simulink model "EMT_ML.before_diagnostic_fixes"  (R2024b)
settings: Solver=ode5  StartTime=0.0  StopTime=200  FixedStep=0.002  RelTol=1e-3
model workspace (MAT data in the model file):
  A = 7.3
  B = 2.71
  C0_shift = 200
  C1_shift = 200
  C2_shift = 200
  Cb = 70
  Cd = 0.6
  EMSInputBus : Simulink.Bus (value not decoded)
  Fb_max = 247500
  JA = 0.4
  JB = 0.4
  JZ = 0.4
  Jc1r2 = 0.01
  Jc3r4 = 0.01
  Jc4 = 0.01
  Je = 2.5
  Jh = 0.01
  Jq1 = 0.01
  Jq2 = 0.01
  Jr1 = 0.01
  Jr3s4 = 0.01
  Js123 = 0.01
  L = 4.472
  NE = [1600 1600 1600 1600 1600 1600 1600 1600 1600 1600 1600 1600 ... (840 elements, 30x28)]
  N_Te = 30
  N_ne = 28
  PE = [0 100.366530527 133.710336161 167.221698607 195.706356687 221.845219395 250.497434286 278.144308305 305.288511886 330.086920096 352.87464656 374.489475338 ... (840 elements, 30x28)]
  PN0 = 0
  Pb_epr = [-45 -45 -40 -30 0 30 40 45 45]
  Pb_max = [0 40 45 45 45]
  Pb_min = [-45 -45 -45 -40 0]
  Pe_ass = 230
  Pe_max = 1103
  Peg = [0 100 120 140 160 180 200 220 240 260 280 300 ... (53 elements, 1x53)]
  R_map = [0.09 0.089 0.09 0.091 0.092 0.093 0.094 0.095 0.096 0.097 0.098]
  SF_C0 = 1.5
  SF_C1 = 1.5
  SF_C2 = 1.5
  SF_Z1 = 1.5
  SF_Z2 = 1.5
  SF_ZD = 1.5
  SOC0 = 60
  SOC_epr = [30 31 50 59 60 61 70 79 80]
  SOC_map = [0 10 20 30 40 50 60 70 80 90 100]
  TA_max_map = [588.855 593.803361345 598.83559322 603.953846154 609.160344828 614.457391304 619.847368421 625.332743363 630.916071429 636.6 642.387272727 648.280733945 ... (115 elements, 1x115)]
  TA_min_map = [-588.855 -593.803361345 -598.83559322 -603.953846154 -609.160344828 -614.457391304 -619.847368421 -625.332743363 -630.916071429 -636.6 -642.387272727 -648.280733945 ... (115 elements, 1x115)]
  TAf = 0
  TB_max_map = [588.855 593.803361345 598.83559322 603.953846154 609.160344828 614.457391304 619.847368421 625.332743363 630.916071429 636.6 642.387272727 648.280733945 ... (115 elements, 1x115)]
  TB_min_map = [-588.855 -593.803361345 -598.83559322 -603.953846154 -609.160344828 -614.457391304 -619.847368421 -625.332743363 -630.916071429 -636.6 -642.387272727 -648.280733945 ... (115 elements, 1x115)]
  TBf = 0
  TE = [0 599 798 998 1168 1324 1495 1660 1822 1970 2106 2235 ... (840 elements, 30x28)]
  TS_A = 0.2
  TS_B = 0.2
  TS_C0 = 0.2
  TS_C1 = 0.2
  TS_C2 = 0.2
  TS_Z = 0.2
  TS_Z1 = 0.2
  TS_Z2 = 0.2
  TS_ZD = 0.2
  TZ_max_map = [537.13125 540.509433962 543.930379747 547.394904459 550.903846154 554.458064516 558.058441558 561.705882353 565.401315789 569.145695364 572.94 576.785234899 ... (131 elements, 1x131)]
  TZ_min_map = [-537.13125 -540.509433962 -543.930379747 -547.394904459 -550.903846154 -554.458064516 -558.058441558 -561.705882353 -565.401315789 -569.145695364 -572.94 -576.785234899 ... (131 elements, 1x131)]
  TZf = 0
  T_generator = [0 185 493.333333333 801.666666667 1110 1418.33333333 1726.66666667]
  T_motor = [0 185 493.333333333 801.666666667 1110 1418.33333333 1726.66666667]
  Te_map = [0 599 798 998 1168 1324 1495 1660 1822 1970 2106 2235 ... (30 elements, 1x30)]
  Te_max = 2754
  Te_max_map = [1168 1324 1495 1660 1822 1970 2106 2235 2355 2458 2543 2606 ... (28 elements, 1x28)]
  Te_start = 1600
  Tef = 100
  Teg = [0 596.8125 636.6 718.741935484 799.916230366 859.41 954.422788606 954.9 996.417391304 1078.98305085 1114.05 1169.26530612 ... (53 elements, 1x53)]
  Temax = 998
  Time = [0 0.1 0.2 0.3 0.4 0.5 0.6 0.7 0.8 0.9 1 1.1 ... (2001 elements, 1x2001)]
  Time_ele = [0 4 8 12 16 20 24 28 32 36 40 44 ... (401 elements, 1x401)]
  Time_fg = [0 2 4 6 8 10 12 14 16 18 20 22 ... (801 elements, 1x801)]
  Tmax_C0 = 2754
  Tmax_C1 = 3505.25455609
  Tmax_C2 = 3505.25455609
  Tmax_Z1 = 5584.80955498
  Tmax_Z2 = 16307.6439005
  Tmax_ZD = 3855.6
  Ts_e = 0.1
  Uoc_map = [814.5 917 933.25 945.75 958.25 969.25 978 985.25 993.25 1003.25 1050]
  V_Shift12 = 32
  V_Shift21 = 25
  V_Start = 10
  Voltage0 = 900
  Voltage_epr = [750 760 900 1000 1050]
  Y_engine = 0.955
  Yc = 0.98
  Yh = 0.96
  Yo = 0.92
  Yq = 0.94
  Z1_shift = 200
  Z2_shift = 200
  a11 = 1.54241568346
  a11_L = 1.54241568346
  a12 = -3.86074191629
  a12_L = 2.43173643789
  a21 = -1.04963112005
  a22 = 2.46948356808
  b11 = 0
  b11_L = 0
  b12 = 3.33
  b12_L = 7.8036
  b21 = 2.23571428571
  b22 = -2.13
  c11 = -0.648333656565
  c12 = 0
  c21 = -0.648333656565
  c22 = 0.680511182109
  controller_id = 1
  controller_name = 'Existing heuristic-grid EMS'
  cycle_grade = [0 0 0 0 0 0 0 0 0 0 0 0 ... (2001 elements, 1x2001)]
  cycle_road = [0.045 0.045 0.045 0.045 0.045 0.045 0.045 0.045 0.045 0.045 0.045 0.045 ... (2001 elements, 1x2001)]
  cycle_steering = [0 0 0 0 0 0 0 0 0 0 0 0 ... (2001 elements, 1x2001)]
  cycle_time = [0 0.1 0.2 0.3 0.4 0.5 0.6 0.7 0.8 0.9 1 1.1 ... (2001 elements, 1x2001)]
  d11 = -0.751666343435
  d12 = 0.3003003003
  d21 = -0.751666343435
  d22 = 0.319488817891
  e11 = -1.54241568346
  e12 = 0
  e21 = 1.04963112005
  e22 = -2.23571428571
  eff_generator = [0.8 0.8 0.79 0.79 0.76 0.74 0.72 0.8 0.85 0.88 0.85 0.8 ... (84 elements, 7x12)]
  eff_motor = [0.8 0.8 0.79 0.79 0.76 0.74 0.72 0.8 0.85 0.88 0.85 0.8 ... (84 elements, 7x12)]
  ele_map = [10 11.46 14.13 19.24 20.94 23.21 20.29 20.23 22.28 17.66 16.24 18.95 ... (401 elements, 1x401)]
  ems_runtime_config : object (value not decoded)
  f11 = -3.86074191629
  f12 = 3.33
  f21 = 2.46948356808
  f22 = -2.13
  fg = 0.045
  fg_map = [0.0125 0.0215 0.0332 0.0452 0.0525 0.0589 0.0584 0.0592 0.0621 0.0576 0.055 0.0572 ... (801 elements, 1x801)]
  fuel_gpkwh = [269.874826377 269.874826377 260.084605263 254.895150301 249.802821062 244.062054381 234.972466555 226.630558735 223.93243551 227.612775381 231.379615385 228.983738255 ... (840 elements, 30x28)]
  fuel_map = [269.874826377 269.874826377 260.084605263 254.895150301 249.802821062 244.062054381 234.972466555 226.630558735 223.93243551 227.612775381 231.379615385 228.983738255 ... (840 elements, 30x28)]
  fuel_map_N = [269.874826377 269.874826377 260.084605263 254.895150301 249.802821062 nan nan nan nan nan nan nan ... (840 elements, 30x28)]
  i = 28
  ic = 4.42
  iq = 1.4
  it = 4
  j = 30
  k1 = 2.13
  k2 = 2.13
  k3 = 2.33
  k4 = 1.92
  kh = 2.88
  kq = 2.17
  kt = 1.83
  mass = 45000
  miu_max = 0.8
  nA_map = [-6000 -5950 -5900 -5850 -5800 -5750 -5700 -5650 -5600 -5550 -5500 -5450 ... (115 elements, 1x115)]
  nA_max = 6000
  nA_min = -6000
  nB_map = [-6000 -5950 -5900 -5850 -5800 -5750 -5700 -5650 -5600 -5550 -5500 -5450 ... (115 elements, 1x115)]
  nB_max = 6000
  nB_min = -6000
  nB_start = 0
  nZ_map = [-8000 -7950 -7900 -7850 -7800 -7750 -7700 -7650 -7600 -7550 -7500 -7450 ... (131 elements, 1x131)]
  nZ_max = 8000
  nZ_min = -8000
  n_generator = [0 318.5 796.25 1274 1751.75 2229.5 2707.25 3185 3662.75 4140.5 4618.25 7007]
  n_motor = [0 318.5 796.25 1274 1751.75 2229.5 2707.25 3185 3662.75 4140.5 4618.25 7007]
  ne_idl = 3000
  ne_map = [1600 1700 1800 1900 2000 2100 2200 2300 2400 2500 2600 2700 ... (28 elements, 1x28)]
  ne_max = 4200
  ne_min = 1600
  ne_start = 200
  neg = [1600 1600 1800 1860 1910 2000 2001 2200 2300 2301 2400 2450 ... (53 elements, 1x53)]
  no_Shift12 = 1589.43589002
  no_Shift21 = 1241.74678908
  rz = 0.318
  startup_feedback_delay_s = 0.002
  startup_power_share = 0.5
  startup_speed_regularizer_rpm = 100
  v_cyc = [0 0 0 0 0 0 0 0 0 0 0 0 ... (2001 elements, 1x2001)]
  voltage_HighA = 1050
  voltage_HighB = 1050
  voltage_HighZ = 1050
  voltage_LowA = 750
  voltage_LowB = 750
  voltage_LowZ = 750
symbols that are objects in the model workspace (value not decoded): ems_runtime_config
undefined symbols (not defined in the file or in its folder): sigbuilder_block
libraries: fl_lib x82, nesl_utility x55, simulink x49, sdl_lib x10, simulink_need_slupdate x6, powerlib_extras x1
(part 3 of 7)

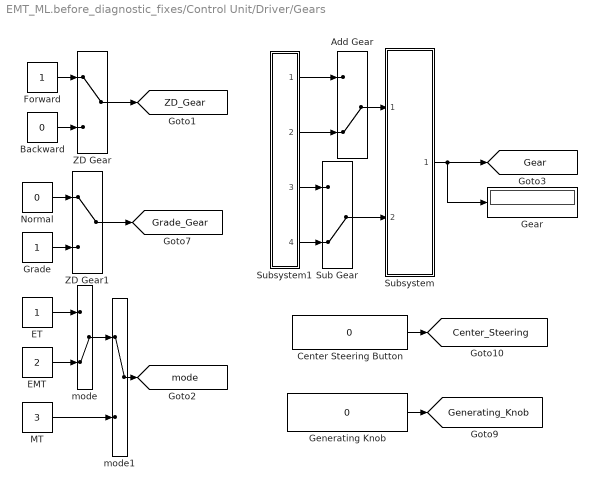
== system EMT_ML.before_diagnostic_fixes/Control Unit/Driver/Gears ==
  "Add Gear " : ManualSwitch  CurrentSetting=0
  Backward : Constant  Value=0
  Center Steering Button : Constant  Value=0
  EMT : Constant  Value=2
  ET : Constant
  Forward : Constant
  Gear : Display
  Generating Knob : Constant  Value=0
  Grade : Constant
  MT : Constant  Value=3
  Normal : Constant  Value=0
  Sub Gear : ManualSwitch  CurrentSetting=0
  Subsystem : Subsystem
  Subsystem1 : Subsystem
  ZD Gear : ManualSwitch
  ZD Gear1 : ManualSwitch
  mode : ManualSwitch  CurrentSetting=0
  mode1 : ManualSwitch
  tag scope: Center_Steering=global, Gear=global, Generating_Knob=global, Grade_Gear=global, ZD_Gear=global, mode=global
  wires:
  ZD Gear1/1 -> [Grade_Gear]
  Normal/1 -> ZD Gear1/1
  Grade/1 -> ZD Gear1/2
  Center Steering Button/1 -> [Center_Steering]
  Generating Knob/1 -> [Generating_Knob]
  mode/1 -> mode1/1
  mode1/1 -> [mode]
  MT/1 -> mode1/2
  EMT/1 -> mode/2
  Subsystem/1(Gear) -> [Gear], Gear/1
  Sub Gear/1 -> Subsystem/2(Sub)
  "Add Gear "/1 -> Subsystem/1(Add)
  Subsystem1/4(4) -> Sub Gear/2
  Subsystem1/3(3) -> Sub Gear/1
  Subsystem1/2(2) -> "Add Gear "/2
  Subsystem1/1(1) -> "Add Gear "/1
  ET/1 -> mode/1
  ZD Gear/1 -> [ZD_Gear]
  Forward/1 -> ZD Gear/1
  Backward/1 -> ZD Gear/2

== system EMT_ML.before_diagnostic_fixes/Control Unit/Driver/Grade Angle ==
  " 0.1" : ManualSwitch  CurrentSetting=0
  10 : ManualSwitch
  Add angle : ManualSwitch
  Forward : Constant  Value=32
  Forward1 : Lookup_n-D  NumberOfTableDimensions=1  BreakpointsForDimension1=cycle_time  Table=cycle_grade  InternalRulePriority=Speed  RndMeth=Simplest
  Forward1_clock : Clock
  Sub angle : ManualSwitch  CurrentSetting=0
  Subsystem4 : Subsystem  mask{Parameter1=on}
      mask prompts: Parameter1 "Pedal"
  Subsystem6 : Subsystem
  Transfer Fcn1 : TransferFcn  Denominator=[0.02 1]
  angle : Display
  tag scope: angle=global
  wires:
  Subsystem4/1(Out1) -> Add angle/1
  Subsystem4/2(Out2) -> Add angle/2
  Subsystem4/3(Out3) -> Sub angle/1
  Add angle/1 -> Subsystem6/1(Add)
  Sub angle/1 -> Subsystem6/2(Sub)
  Subsystem4/4(Out4) -> Sub angle/2
  Subsystem4/5(Out5) -> " 0.1"/1
  Subsystem4/6(Out6) -> " 0.1"/2
  Subsystem4/7(Out7) -> 10/1
  Subsystem4/8(Out8) -> 10/2
  " 0.1"/1 -> Subsystem6/3(0.1)
  10/1 -> Subsystem6/4(10)
  Subsystem6/1(angle) -> Transfer Fcn1/1, angle/1
  Forward1_clock/1 -> Forward1/1
  Forward1/1 -> [angle]

== system EMT_ML.before_diagnostic_fixes/Control Unit/Driver/Ground Resistance Coefficient ==
  *0.1 : ManualSwitch
  *10 : ManualSwitch
  Add : Sum
  Add fg : ManualSwitch  CurrentSetting=0
  Add1 : Sum
  Forward : Constant  Value=0.07
  Forward1 : Lookup_n-D  NumberOfTableDimensions=1  BreakpointsForDimension1=cycle_time  Table=cycle_road  InternalRulePriority=Speed  RndMeth=Simplest
  Forward1_clock : Clock
  Road : Subsystem
  Road1 : Subsystem
  Saturation : Saturate  UpperLimit=0.6  LowerLimit=0.04
  Saturation1 : Saturate  UpperLimit=0.6  LowerLimit=0.04
  Sub fg : ManualSwitch  CurrentSetting=0
  Subsystem2 : Subsystem  mask{Parameter1=on}
      mask prompts: Parameter1 "Pedal"
  Subsystem3 : Subsystem
  Transfer Fcn1 : TransferFcn  Denominator=[0.02 1]
  Uniform Random Number : UniformRandomNumber  Minimum=-0.01  Maximum=0.01  SampleTime=1
  fg : Display
  tag scope: fg_act=global
  wires:
  Road/1(fg) -> Add/2
  Subsystem3/1(fg) -> Add/1
  Subsystem2/1(Out1) -> Add fg/1
  Subsystem2/2(Out2) -> Add fg/2
  Subsystem2/3(Out3) -> Sub fg/1
  Add fg/1 -> Subsystem3/1(Add)
  Sub fg/1 -> Subsystem3/2(Sub)
  Subsystem2/4(Out4) -> Sub fg/2
  Subsystem2/5(Out5) -> *0.1/1
  Subsystem2/6(Out6) -> *0.1/2
  Subsystem2/7(Out7) -> *10/1
  Subsystem2/8(Out8) -> *10/2
  *0.1/1 -> Subsystem3/3(0.1)
  *10/1 -> Subsystem3/4(10)
  Transfer Fcn1/1 -> fg/1
  Add/1 -> Saturation/1
  Uniform Random Number/1 -> Add1/2
  Road1/1(fg) -> Saturation1/1
  Forward/1 -> Add1/1
  Add1/1 -> Transfer Fcn1/1
  Forward1_clock/1 -> Forward1/1
  Forward1/1 -> [fg_act]

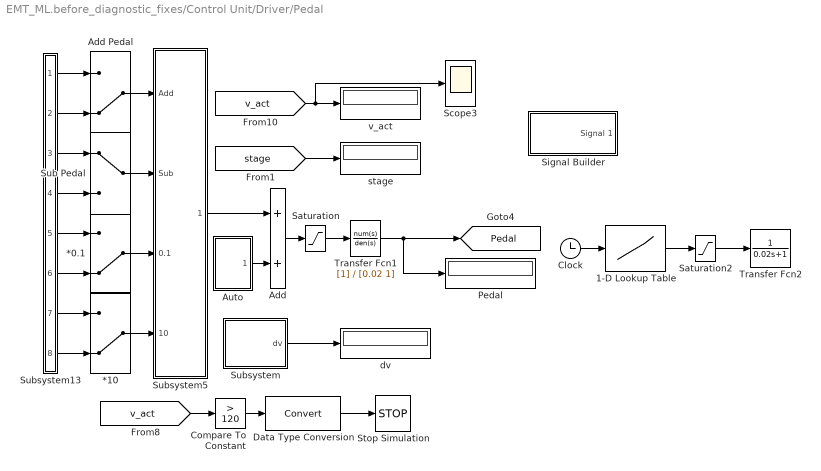
== system EMT_ML.before_diagnostic_fixes/Control Unit/Driver/Pedal  ==
  *0.1 : ManualSwitch  CurrentSetting=0
  *10 : ManualSwitch  CurrentSetting=0
  1-D Lookup Table : Lookup_n-D  NumberOfTableDimensions=1  BreakpointsForDimension1=[0 100 101 200]  Table=[1 1 -1 -1]  RndMeth=Simplest
  Add : Sum
  Add Pedal : ManualSwitch  CurrentSetting=0
  Auto : Subsystem
  Clock : Clock
  Compare To Constant : simulink/Logic and Bit Operations/Compare To Constant  relop=>  const=120  OutDataTypeStr=uint8
  Data Type Conversion : DataTypeConversion  SaturateOnIntegerOverflow=off  RndMeth=Floor
  Pedal : Display
  Saturation : Saturate  UpperLimit=1  LowerLimit=-1
  Saturation2 : Saturate  UpperLimit=1  LowerLimit=-1
  Scope3 : Scope
  Signal Builder : Subsystem  Tag=STV Subsys  LoadFcn=sigbuilder_block('load');  StartFcn=sigbuilder_block('start');  StopFcn=sigbuilder_block('stop');  ClipboardFcn=sigbuilder_block('clipboard');  mask(Sigbuilder block){tuvar=[0:10]}
      mask help: Simulink:masks:SigbuilderBlock_MD
      mask init:
      | if ~strcmp(get_param(bdroot(gcbh),'SimulationStatus'),'stopped') tuvar = sigbuilder_block('maskInit'); end
      settings: CopyFcn=sigbuilder_block('copy');  DeleteFcn=sigbuilder_block('delete');  ModelCloseFcn=sigbuilder_block('modelClose');  PreSaveFcn=sigbuilder_block('preSave');  PauseFcn=sigbuilder_block('pause')  ContinueFcn=sigbuilder_block('continue')  NameChangeFcn=sigbuilder_block('namechange');  OpenFcn=sigbuilder_block('open',[437.25 199.5 550.5 399.75 ]);  CloseFcn=sigbuilder_block('close');
      mask Display: plot(0, 0, 100, 100,[2, 2, 32, 32, 2], [68, 8, 8, 68, 68],[32, 2], [38, 38], [32, 19, 2],[53, 60, 44], [32, 17, 17, 2],[16, 16, 31, 31]);txt = getActiveGroup(gcbh);text(2, 100, txt,'verticalAlignment', 'top');
  Stop Simulation : Stop
  Sub Pedal : ManualSwitch
  Subsystem : Subsystem
  Subsystem13 : Subsystem  mask{Parameter1=on}
      mask prompts: Parameter1 "Pedal"
  Subsystem5 : Subsystem
  Transfer Fcn1 : TransferFcn  Denominator=[0.02 1]
  Transfer Fcn2 : TransferFcn  Denominator=[0.02 1]
  dv : Display
  stage : Display
  v_act : Display
  tag scope: Pedal=global
  wires:
  Subsystem5/1(Pedal) -> Add/1
  Subsystem/1(dv) -> dv/1
  [stage] -> stage/1
  [v_act] -> Scope3/1, v_act/1
  *10/1 -> Subsystem5/4(10)
  *0.1/1 -> Subsystem5/3(0.1)
  Subsystem13/8(Out8) -> *10/2
  Subsystem13/7(Out7) -> *10/1
  Subsystem13/6(Out6) -> *0.1/2
  Subsystem13/5(Out5) -> *0.1/1
  Subsystem13/4(Out4) -> Sub Pedal/2
  Sub Pedal/1 -> Subsystem5/2(Sub)
  Add Pedal/1 -> Subsystem5/1(Add)
  Subsystem13/3(Out3) -> Sub Pedal/1
  Subsystem13/2(Out2) -> Add Pedal/2
  Subsystem13/1(Out1) -> Add Pedal/1
  [v_act] -> Compare To Constant/1
  Compare To Constant/1 -> Data Type Conversion/1
  Data Type Conversion/1 -> Stop Simulation/1
  Saturation/1 -> Transfer Fcn1/1
  Add/1 -> Saturation/1
  Clock/1 -> 1-D Lookup Table/1
  1-D Lookup Table/1 -> Saturation2/1
  Saturation2/1 -> Transfer Fcn2/1
  Auto/1(Pedal) -> Add/2
  Transfer Fcn1/1 -> Pedal/1, [Pedal]

== system EMT_ML.before_diagnostic_fixes/Control Unit/Driver/Wheel Angle ==
  " x 0.1" : ManualSwitch  CurrentSetting=0
  Add wheel : ManualSwitch
  Sub Wheel : ManualSwitch  CurrentSetting=0
  Subsystem1 : Subsystem  mask{Parameter1=on}
      mask prompts: Parameter1 "Pedal"
  Subsystem2 : Subsystem
  Wheel : Display
  x10 : ManualSwitch
  tag scope: Wheel=global
  wires:
  Subsystem2/1(wheel) -> Wheel/1, [Wheel]
  Subsystem1/1(Out1) -> Add wheel/1
  Subsystem1/2(Out2) -> Add wheel/2
  Subsystem1/3(Out3) -> Sub Wheel/1
  Add wheel/1 -> Subsystem2/1(Add)
  Sub Wheel/1 -> Subsystem2/2(Sub)
  Subsystem1/4(Out4) -> Sub Wheel/2
  Subsystem1/5(Out5) -> " x 0.1"/1
  Subsystem1/6(Out6) -> " x 0.1"/2
  Subsystem1/7(Out7) -> x10/1
  Subsystem1/8(Out8) -> x10/2
  " x 0.1"/1 -> Subsystem2/3(0.1)
  x10/1 -> Subsystem2/4(10)

== system EMT_ML.before_diagnostic_fixes/Front Gear/C0/C0 ==
  Press : Inport
  C0 : sdl_lib/Clutches/Disc Friction Clutch  geometry_model=2  r_eff=130 mm  d_o=145*2 mm  d_i=110*2 mm  nS=6  piston_area=0.0347 m^2  unidirectional=0  friction_model=1  mu_w_vector=[ 0 0.1 0.2 0.3 0.4 0.5 1 2 5 10 100 1000 ] rad/s  temperature_TLU=[280.0, 300.0, 320.0] K  mu_static=0.10  mu_static_vector=[0.4, 0.38, 0.36]  mu_coulomb=0.06  mu_coulomb_vector=[ 0.29 0.28 0.26 0.22 0.21 0.2 0.2 0.19 0.19 0.19 0.19 0.19 ]  mu_coulomb_temp_vector=[0.3, 0.28, 0.25]  mu_coulomb_matrix=[0.34, 0.32, 0.3; 0.3, 0.28, 0.25; 0.25, 0.2, 0.15]  mu_interp_method=1  mu_extrap_method=1  d_f=0.6  w_tol=0.001 rad/s  pressure_min=1560 Pa  mu_visc=0.0256 N*m/(rad/s)  initial_state_locked=1  thermal_mass=25 kJ/K  T_init=300 K
      settings: InternalSimscapePortConfiguration="{\"Bottom\":[],\"Left\":[{\"id\":\"P\",\"label\":\"P\",\"type\":\"input\"},{\"id\":\"B\",\"label\":\"B\",\"type\":\"foundation.mechanical.rotational.rotational\"}],\"Right\":[{\"id\":\"F\",\"label\":\"F\",\"type\":\"foundation.mechanical.rotational.rotational\"}],\"Top\":[]}"
  Simulink-PS Converter : nesl_utility/Simulink-PS Converter  PhysicalDomain=network_engine_domain  SubClassName=ps_input  LeftPortType=input  RightPortType=output  PseudoPeriodic=off  Frequencies=[]  NoiseDistribution=none  NoiseParameters=[]  Unit=Pa  AffineConversion=off  FilteringAndDerivatives=filter  SimscapeFilterOrder=1  InputFilterTimeConstant=.001  UdotUserProvided=1
  Slip Sensor : Subsystem  mask(Slip Sensor){}
      mask help: The speed unit is r/min.
  Tire Radius2 : Gain  Gain=2500000
  In : PMIOPort  Side=Left
  Out : PMIOPort  Port=2  Side=Right
  r/min : Outport
  wires:
  Slip Sensor/1(r/min) -> r/min/1
  Press/1 -> Tire Radius2/1
  Tire Radius2/1 -> Simulink-PS Converter/1
  connections:
  Slip Sensor/LConn1 -- C0/LConn2 -- In/RConn1
  Slip Sensor/RConn1 -- C0/RConn1 -- Out/RConn1
  Simulink-PS Converter/RConn1 -- C0/LConn1

== system EMT_ML.before_diagnostic_fixes/Front Gear/C0/Power ==
  Gain1 : Gain  Gain=1/9549
  Product3 : Product  RndMeth=Zero
  Speed Sensor : Subsystem  mask(Speed Sensor){}
      mask help: The speed unit is r/min.
  Torque Sensor : Subsystem  mask(Torque Sensor){}
      mask help: The torque unit is Nm.
  In : PMIOPort  Side=Left
  Out : PMIOPort  Port=2  Side=Right
  kW : Outport
  wires:
  Speed Sensor/1(r/min) -> Product3/2
  Torque Sensor/1(Nm) -> Gain1/1
  Gain1/1 -> Product3/1
  Product3/1 -> kW/1
  connections:
  Out/RConn1 -- Torque Sensor/RConn1 -- Speed Sensor/LConn1
  In/RConn1 -- Torque Sensor/LConn1

== system EMT_ML.before_diagnostic_fixes/Front Gear/C0/Power1 ==
  Gain1 : Gain  Gain=1/9549
  Product3 : Product  RndMeth=Zero
  Speed Sensor : Subsystem  mask(Speed Sensor){}
      mask help: The speed unit is r/min.
  Torque Sensor : Subsystem  mask(Torque Sensor){}
      mask help: The torque unit is Nm.
  In : PMIOPort  Side=Left
  Out : PMIOPort  Port=2  Side=Right
  kW : Outport
  wires:
  Product3/1 -> kW/1
  Gain1/1 -> Product3/1
  Torque Sensor/1(Nm) -> Gain1/1
  Speed Sensor/1(r/min) -> Product3/2
  connections:
  In/RConn1 -- Torque Sensor/LConn1
  Torque Sensor/RConn1 -- Out/RConn1 -- Speed Sensor/LConn1

== system EMT_ML.before_diagnostic_fixes/Front Gear/Subsystem/Speed Sensor ==
  Ideal Rotational Motion Sensor : fl_lib/Mechanical/Mechanical Sensors/Ideal Rotational Motion Sensor  reference=foundation.enum.MeasurementReference.difference  acceleration_port=false  velocity_port=true  position_port=true  wrap_angle=false  offset=0 rad
  PS-Simulink Converter : nesl_utility/PS-Simulink Converter  PhysicalDomain=network_engine_domain  SubClassName=ps_output  LeftPortType=input  RightPortType=output  PseudoPeriodic=off  Frequencies=[]  VectorFormat=1-D array  Unit=rad/s  AffineConversion=off
  Reference : fl_lib/Mechanical/Rotational Elements/Mechanical Rotational Reference
  Tire Radius2 : Gain  Gain=30/pi
  shaft : PMIOPort  Side=Left
  r/min : Outport
  wires:
  Tire Radius2/1 -> r/min/1
  PS-Simulink Converter/1 -> Tire Radius2/1
  connections:
  shaft/RConn1 -- Ideal Rotational Motion Sensor/LConn1
  Reference/LConn1 -- Ideal Rotational Motion Sensor/RConn1
  PS-Simulink Converter/LConn1 -- Ideal Rotational Motion Sensor/RConn2

== system EMT_ML.before_diagnostic_fixes/Front Gear/Subsystem/Torque Sensor ==
  Ideal Torque Sensor : fl_lib/Mechanical/Mechanical Sensors/Ideal Torque Sensor
  PS-Simulink Converter : nesl_utility/PS-Simulink Converter  PhysicalDomain=network_engine_domain  SubClassName=ps_output  LeftPortType=input  RightPortType=output  PseudoPeriodic=off  Frequencies=[]  VectorFormat=1-D array  Unit=1  AffineConversion=off
  In : PMIOPort  Side=Left
  Out : PMIOPort  Port=2  Side=Right
  Nm : Outport
  wires:
  PS-Simulink Converter/1 -> Nm/1
  connections:
  PS-Simulink Converter/LConn1 -- Ideal Torque Sensor/RConn2
  In/RConn1 -- Ideal Torque Sensor/LConn1
  Ideal Torque Sensor/RConn1 -- Out/RConn1

== system EMT_ML.before_diagnostic_fixes/Power Coupler /C1/C2 ==
  Press : Inport
  C1 : sdl_lib/Clutches/Disc Friction Clutch  geometry_model=2  r_eff=130 mm  d_o=167*2 mm  d_i=143*2 mm  nS=8  piston_area=0.0290 m^2  unidirectional=0  friction_model=1  mu_w_vector=[ 0 0.1 0.2 0.3 0.4 0.5 1 2 5 10 100 1000 ] rad/s  temperature_TLU=[280.0, 300.0, 320.0] K  mu_static=0.10  mu_static_vector=[0.4, 0.38, 0.36]  mu_coulomb=0.06  mu_coulomb_vector=[ 0.29 0.28 0.26 0.22 0.21 0.2 0.2 0.19 0.19 0.19 0.19 0.19 ]  mu_coulomb_temp_vector=[0.3, 0.28, 0.25]  mu_coulomb_matrix=[0.34, 0.32, 0.3; 0.3, 0.28, 0.25; 0.25, 0.2, 0.15]  mu_interp_method=1  mu_extrap_method=1  d_f=0.6  w_tol=0.001 rad/s  pressure_min=1840 Pa  mu_visc=0.0414 N*m/(rad/s)  initial_state_locked=0  thermal_mass=25 kJ/K  T_init=300 K
      settings: InternalSimscapePortConfiguration="{\"Bottom\":[],\"Left\":[{\"id\":\"P\",\"label\":\"P\",\"type\":\"input\"},{\"id\":\"B\",\"label\":\"B\",\"type\":\"foundation.mechanical.rotational.rotational\"}],\"Right\":[{\"id\":\"F\",\"label\":\"F\",\"type\":\"foundation.mechanical.rotational.rotational\"}],\"Top\":[]}"
  Simulink-PS Converter : nesl_utility/Simulink-PS Converter  PhysicalDomain=network_engine_domain  SubClassName=ps_input  LeftPortType=input  RightPortType=output  PseudoPeriodic=off  Frequencies=[]  NoiseDistribution=none  NoiseParameters=[]  Unit=Pa  AffineConversion=off  FilteringAndDerivatives=filter  SimscapeFilterOrder=1  InputFilterTimeConstant=.001  UdotUserProvided=1
  Slip Sensor : Subsystem  mask(Slip Sensor){}
      mask help: The speed unit is r/min.
  Tire Radius2 : Gain  Gain=2500000
  In : PMIOPort  Side=Left
  Out : PMIOPort  Port=2  Side=Right
  r/min : Outport
  wires:
  Tire Radius2/1 -> Simulink-PS Converter/1
  Press/1 -> Tire Radius2/1
  Slip Sensor/1(r/min) -> r/min/1
  connections:
  Simulink-PS Converter/RConn1 -- C1/LConn1
  In/RConn1 -- C1/LConn2 -- Slip Sensor/LConn1
  C1/RConn1 -- Out/RConn1 -- Slip Sensor/RConn1

== system EMT_ML.before_diagnostic_fixes/Power Coupler /C1/Power ==
  Gain1 : Gain  Gain=1/9549
  Product3 : Product  RndMeth=Zero
  Speed Sensor : Subsystem  mask(Speed Sensor){}
      mask help: The speed unit is r/min.
  Torque Sensor : Subsystem  mask(Torque Sensor){}
      mask help: The torque unit is Nm.
  In : PMIOPort  Side=Left
  Out : PMIOPort  Port=2  Side=Right
  kW : Outport
  wires:
  Product3/1 -> kW/1
  Gain1/1 -> Product3/1
  Torque Sensor/1(Nm) -> Gain1/1
  Speed Sensor/1(r/min) -> Product3/2
  connections:
  In/RConn1 -- Torque Sensor/LConn1
  Torque Sensor/RConn1 -- Out/RConn1 -- Speed Sensor/LConn1

== system EMT_ML.before_diagnostic_fixes/Power Coupler /C1/Power1 ==
  Gain1 : Gain  Gain=1/9549
  Product3 : Product  RndMeth=Zero
  Speed Sensor : Subsystem  mask(Speed Sensor){}
      mask help: The speed unit is r/min.
  Torque Sensor : Subsystem  mask(Torque Sensor){}
      mask help: The torque unit is Nm.
  In : PMIOPort  Side=Left
  Out : PMIOPort  Port=2  Side=Right
  kW : Outport
  wires:
  Speed Sensor/1(r/min) -> Product3/2
  Torque Sensor/1(Nm) -> Gain1/1
  Gain1/1 -> Product3/1
  Product3/1 -> kW/1
  connections:
  Speed Sensor/LConn1 -- Out/RConn1 -- Torque Sensor/RConn1
  In/RConn1 -- Torque Sensor/LConn1

== system EMT_ML.before_diagnostic_fixes/Power Coupler /Z1/Z ==
  Abs : Abs  SaturateOnIntegerOverflow=off
  Add : Sum  Inputs=+-
  Power : Subsystem
  Power1 : Subsystem
  Z1 : Subsystem
  In : PMIOPort  Side=Left
  Out : PMIOPort  Port=2  Side=Right
  tag scope: Z1_loss=global, Z1_rela=global
  wires:
  Z1/1(r/min) -> [Z1_rela]
  [Press_Z1] -> Z1/1(Press)
  Power1/1(kW) -> Add/2
  Power/1(kW) -> Add/1
  Abs/1 -> [Z1_loss]
  Add/1 -> Abs/1
  connections:
  In/RConn1 -- Power/LConn1
  Power/RConn1 -- Z1/LConn1
  Z1/RConn1 -- Power1/LConn1
  Power1/RConn1 -- Out/RConn1

== system EMT_ML.before_diagnostic_fixes/Power Coupler /Z2/Z ==
  Abs : Abs  SaturateOnIntegerOverflow=off
  Add : Sum  Inputs=+-
  Power : Subsystem
  Power1 : Subsystem
  Z2 : Subsystem
  In : PMIOPort  Side=Left
  Out : PMIOPort  Port=2  Side=Right
  tag scope: Z2_loss=global, Z2_rela=global
  wires:
  [Press_Z2] -> Z2/1(Press)
  Z2/1(r/min) -> [Z2_rela]
  Add/1 -> Abs/1
  Abs/1 -> [Z2_loss]
  Power1/1(kW) -> Add/2
  Power/1(kW) -> Add/1
  connections:
  In/RConn1 -- Power/LConn1
  Power/RConn1 -- Z2/LConn1
  Z2/RConn1 -- Power1/LConn1
  Power1/RConn1 -- Out/RConn1

== system EMT_ML.before_diagnostic_fixes/Rear Gear/Subsystem/Speed Sensor ==
  Ideal Rotational Motion Sensor : fl_lib/Mechanical/Mechanical Sensors/Ideal Rotational Motion Sensor  reference=foundation.enum.MeasurementReference.difference  acceleration_port=false  velocity_port=true  position_port=true  wrap_angle=false  offset=0 rad
  PS-Simulink Converter : nesl_utility/PS-Simulink Converter  PhysicalDomain=network_engine_domain  SubClassName=ps_output  LeftPortType=input  RightPortType=output  PseudoPeriodic=off  Frequencies=[]  VectorFormat=1-D array  Unit=rad/s  AffineConversion=off
  Reference : fl_lib/Mechanical/Rotational Elements/Mechanical Rotational Reference
  Tire Radius2 : Gain  Gain=30/pi
  shaft : PMIOPort  Side=Left
  r/min : Outport
  wires:
  Tire Radius2/1 -> r/min/1
  PS-Simulink Converter/1 -> Tire Radius2/1
  connections:
  shaft/RConn1 -- Ideal Rotational Motion Sensor/LConn1
  Reference/LConn1 -- Ideal Rotational Motion Sensor/RConn1
  PS-Simulink Converter/LConn1 -- Ideal Rotational Motion Sensor/RConn2

== system EMT_ML.before_diagnostic_fixes/Rear Gear/Subsystem/Torque Sensor ==
  Ideal Torque Sensor : fl_lib/Mechanical/Mechanical Sensors/Ideal Torque Sensor
  PS-Simulink Converter : nesl_utility/PS-Simulink Converter  PhysicalDomain=network_engine_domain  SubClassName=ps_output  LeftPortType=input  RightPortType=output  PseudoPeriodic=off  Frequencies=[]  VectorFormat=1-D array  Unit=1  AffineConversion=off
  In : PMIOPort  Side=Left
  Out : PMIOPort  Port=2  Side=Right
  Nm : Outport
  wires:
  PS-Simulink Converter/1 -> Nm/1
  connections:
  PS-Simulink Converter/LConn1 -- Ideal Torque Sensor/RConn2
  In/RConn1 -- Ideal Torque Sensor/LConn1
  Ideal Torque Sensor/RConn1 -- Out/RConn1

== system EMT_ML.before_diagnostic_fixes/Simulation Results/Engine Viewer/Fuel  ==
  FuelConsumption : Lookup2D  RowIndex=ne_map  ColumnIndex=Te_map  Table=fuel_map'  LookUpMeth=Interpolation-Use End Values  SaturateOnIntegerOverflow=off  InputSameDT=off
  Gain : Gain  Gain=1/3600/0.84/1000
  Gain1 : Gain  Gain=1/9549
  Integrator : Integrator  IgnoreLimit=on
  Product1 : Product  RndMeth=Zero
  Product2 : Product  RndMeth=Zero
  Product3 : Product  RndMeth=Zero
  Saturation : Saturate  UpperLimit=max(ne_map)  LowerLimit=min(ne_map)
  Saturation1 : Saturate  UpperLimit=max(Te_map)  LowerLimit=min(Te_map)
  Saturation2 : Saturate  UpperLimit=max(ne_map)*max(Te_map)/9549  LowerLimit=0
  fuel_L : Outport
  gpkWh : Outport  Port=2
  tag scope: eng_fuel_gpkWh=global, fuel_L=global
  wires:
  [Te_act] -> Product1/2, Saturation1/1
  [ne_act] -> Product1/1, Saturation/1
  Saturation2/1 -> Product3/2
  Gain1/1 -> Saturation2/1
  Saturation1/1 -> FuelConsumption/2
  Gain/1 -> Integrator/1
  Integrator/1 -> [fuel_L], fuel_L/1
  Product3/1 -> Gain/1
  Saturation/1 -> FuelConsumption/1
  Product1/1 -> Gain1/1
  Product2/1 -> Product3/1, [eng_fuel_gpkWh], gpkWh/1
  [engine_switch] -> Product2/1
  FuelConsumption/1 -> Product2/2

== system EMT_ML.before_diagnostic_fixes/Simulation Results/Vehicle Viewer/Subsystem1 ==
  0 : Inport
  Constant : Constant  Value=0.001
  MinMax : MinMax  Function=max  Inputs=2
  1 : Outport
  wires:
  MinMax/1 -> 1/1
  0/1 -> MinMax/1
  Constant/1 -> MinMax/2

== system EMT_ML.before_diagnostic_fixes/Simulation Results/Vehicle Viewer/Subsystem7 ==
  0 : Inport
  Constant : Constant  Value=0
  MinMax : MinMax  Function=max  Inputs=2
  1 : Outport
  wires:
  Constant/1 -> MinMax/2
  0/1 -> MinMax/1
  MinMax/1 -> 1/1

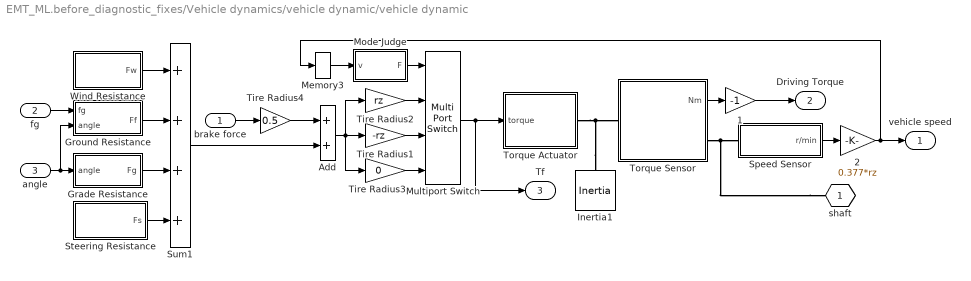
== system EMT_ML.before_diagnostic_fixes/Vehicle dynamics/vehicle dynamic/vehicle dynamic ==
  brake force : Inport
  fg : Inport  Port=2
  angle : Inport  Port=3
  1 : Gain  Gain=-1
  2 : Gain  Gain=0.377*rz
  Add : Sum
  Grade Resistance : Subsystem
  Ground Resistance : Subsystem
  Inertia1 : fl_lib/Mechanical/Rotational Elements/Inertia  inertia=0.5*mass*rz^2 kg*m^2  num_ports=foundation.enum.numPorts2.one  w_specify=on  w_priority=High  w=0 rad/s  w_nominal_specify=off  w_nominal_value=1  w_nominal_unit=rad/s  t_specify=off  t_priority=None  t=0 N*m  t_nominal_specify=off  t_nominal_value=1  t_nominal_unit=N*m
  Memory3 : Memory
  Mode Judge : Subsystem
  Multiport Switch : MultiPortSwitch  SaturateOnIntegerOverflow=off  InputSameDT=off
  Speed Sensor : Subsystem  mask(Speed Sensor){}
      mask help: The speed unit is r/min.
  Steering Resistance : Subsystem
  Sum1 : Sum  Inputs=++++
  Tire Radius1 : Gain  Gain=-rz
  Tire Radius2 : Gain  Gain=rz
  Tire Radius3 : Gain  Gain=0
  Tire Radius4 : Gain  Gain=0.5
  Torque Actuator : Subsystem  mask(Torque Actuator){}
      mask help: The torque unit is Nm.
  Torque Sensor : Subsystem  mask(Torque Sensor){}
      mask help: The torque unit is Nm.
  Wind Resistance : Subsystem
  shaft : PMIOPort  Side=Left
  vehicle speed : Outport
  Driving Torque : Outport  Port=2
  Tf : Outport  Port=3
  wires:
  Tire Radius3/1 -> Multiport Switch/4
  Add/1 -> Tire Radius3/1, Tire Radius1/1, Tire Radius2/1
  Tire Radius1/1 -> Multiport Switch/3
  Tire Radius2/1 -> Multiport Switch/2
  Mode Judge/1(F) -> Multiport Switch/1
  1/1 -> Driving Torque/1
  Torque Sensor/1(Nm) -> 1/1
  Sum1/1 -> Add/2
  2/1 -> vehicle speed/1, Memory3/1
  brake force/1 -> Tire Radius4/1
  Speed Sensor/1(r/min) -> 2/1
  Ground Resistance/1(Ff) -> Sum1/2
  Wind Resistance/1(Fw) -> Sum1/1
  Tire Radius4/1 -> Add/1
  Steering Resistance/1(Fs) -> Sum1/4
  Grade Resistance/1(Fg) -> Sum1/3
  Memory3/1 -> Mode Judge/1(v)
  Multiport Switch/1 -> Torque Actuator/1(torque), Tf/1
  angle/1 -> Grade Resistance/1(angle), Ground Resistance/2(angle)
  fg/1 -> Ground Resistance/1(fg)
  connections:
  shaft/RConn1 -- Speed Sensor/LConn1 -- Torque Sensor/RConn1
  Inertia1/LConn1 -- Torque Actuator/RConn1 -- Torque Sensor/LConn1

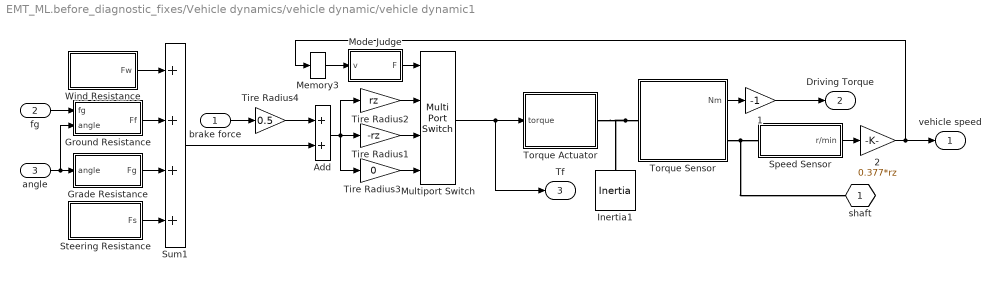
== system EMT_ML.before_diagnostic_fixes/Vehicle dynamics/vehicle dynamic/vehicle dynamic1 ==
  brake force : Inport
  fg : Inport  Port=2
  angle : Inport  Port=3
  1 : Gain  Gain=-1
  2 : Gain  Gain=0.377*rz
  Add : Sum
  Grade Resistance : Subsystem
  Ground Resistance : Subsystem
  Inertia1 : fl_lib/Mechanical/Rotational Elements/Inertia  inertia=0.5*mass*rz^2 kg*m^2  num_ports=foundation.enum.numPorts2.one  w_specify=on  w_priority=High  w=0 rad/s  w_nominal_specify=off  w_nominal_value=1  w_nominal_unit=rad/s  t_specify=off  t_priority=None  t=0 N*m  t_nominal_specify=off  t_nominal_value=1  t_nominal_unit=N*m
  Memory3 : Memory
  Mode Judge : Subsystem
  Multiport Switch : MultiPortSwitch  SaturateOnIntegerOverflow=off  InputSameDT=off
  Speed Sensor : Subsystem  mask(Speed Sensor){}
      mask help: The speed unit is r/min.
  Steering Resistance : Subsystem
  Sum1 : Sum  Inputs=++++
  Tire Radius1 : Gain  Gain=-rz
  Tire Radius2 : Gain  Gain=rz
  Tire Radius3 : Gain  Gain=0
  Tire Radius4 : Gain  Gain=0.5
  Torque Actuator : Subsystem  mask(Torque Actuator){}
      mask help: The torque unit is Nm.
  Torque Sensor : Subsystem  mask(Torque Sensor){}
      mask help: The torque unit is Nm.
  Wind Resistance : Subsystem
  shaft : PMIOPort  Side=Left
  vehicle speed : Outport
  Driving Torque : Outport  Port=2
  Tf : Outport  Port=3
  wires:
  Memory3/1 -> Mode Judge/1(v)
  Grade Resistance/1(Fg) -> Sum1/3
  Steering Resistance/1(Fs) -> Sum1/4
  Tire Radius4/1 -> Add/1
  Wind Resistance/1(Fw) -> Sum1/1
  Ground Resistance/1(Ff) -> Sum1/2
  Speed Sensor/1(r/min) -> 2/1
  brake force/1 -> Tire Radius4/1
  2/1 -> vehicle speed/1, Memory3/1
  Sum1/1 -> Add/2
  Torque Sensor/1(Nm) -> 1/1
  1/1 -> Driving Torque/1
  Mode Judge/1(F) -> Multiport Switch/1
  Tire Radius2/1 -> Multiport Switch/2
  Tire Radius1/1 -> Multiport Switch/3
  Add/1 -> Tire Radius2/1, Tire Radius1/1, Tire Radius3/1
  Tire Radius3/1 -> Multiport Switch/4
  Multiport Switch/1 -> Torque Actuator/1(torque), Tf/1
  angle/1 -> Ground Resistance/2(angle), Grade Resistance/1(angle)
  fg/1 -> Ground Resistance/1(fg)
  connections:
  Torque Sensor/LConn1 -- Torque Actuator/RConn1 -- Inertia1/LConn1
  Torque Sensor/RConn1 -- Speed Sensor/LConn1 -- shaft/RConn1

== system EMT_ML.before_diagnostic_fixes/engine/Engine/Speed Sensor ==
  Ideal Rotational Motion Sensor : fl_lib/Mechanical/Mechanical Sensors/Ideal Rotational Motion Sensor  reference=foundation.enum.MeasurementReference.difference  acceleration_port=false  velocity_port=true  position_port=true  wrap_angle=false  offset=0 rad
  PS-Simulink Converter : nesl_utility/PS-Simulink Converter  PhysicalDomain=network_engine_domain  SubClassName=ps_output  LeftPortType=input  RightPortType=output  PseudoPeriodic=off  Frequencies=[]  VectorFormat=1-D array  Unit=rad/s  AffineConversion=off
  Reference : fl_lib/Mechanical/Rotational Elements/Mechanical Rotational Reference
  Tire Radius2 : Gain  Gain=30/pi
  shaft : PMIOPort  Side=Left
  r/min : Outport
  wires:
  Tire Radius2/1 -> r/min/1
  PS-Simulink Converter/1 -> Tire Radius2/1
  connections:
  shaft/RConn1 -- Ideal Rotational Motion Sensor/LConn1
  Reference/LConn1 -- Ideal Rotational Motion Sensor/RConn1
  PS-Simulink Converter/LConn1 -- Ideal Rotational Motion Sensor/RConn2

== system EMT_ML.before_diagnostic_fixes/engine/Engine/Subsystem ==
  ne_act : Inport
  Te_com : Inport  Port=2
  switch : Inport  Port=3
  Constant1 : Constant  Value=0
  Fcn : Fcn  Expr=u*(1103-180)/1103
  Lookup Table : Lookup  InputValues=ne_map  Table=Te_max_map  SaturateOnIntegerOverflow=off
  Product : Product  RndMeth=Zero
  Saturation : Saturate  UpperLimit=max(ne_map)  LowerLimit=min(ne_map)
  Saturation Dynamic : simulink/Discontinuities/Saturation Dynamic  OutMin=[]  OutMax=[]  OutDataTypeStr=Inherit: Same as second input  OutDataType=sfix(16)  OutScaling=2^-10  DoSatur=off
  Tire Radius2 : Gain  Gain=Y_engine
  Transfer Fcn1 : TransferFcn  Denominator=[T 1]
  Te_act : Outport
  Torque : Outport  Port=2
  wires:
  Transfer Fcn1/1 -> Product/1
  switch/1 -> Product/2
  Saturation Dynamic/1 -> Transfer Fcn1/1
  Saturation/1 -> Lookup Table/1
  Lookup Table/1 -> Saturation Dynamic/1
  Constant1/1 -> Saturation Dynamic/3
  Product/1 -> Tire Radius2/1, Te_act/1
  ne_act/1 -> Saturation/1
  Te_com/1 -> Saturation Dynamic/2
  Tire Radius2/1 -> Fcn/1
  Fcn/1 -> Torque/1

== system EMT_ML.before_diagnostic_fixes/engine/Engine/Subsystem1 ==
  ne : Inport
  Abs1 : Abs  SaturateOnIntegerOverflow=off
  Constant1 : Constant  Value=0
  Constant2 : Constant  Value=-Tef
  Constant3 : Constant  Value=-Te_start
  Constant5 : Constant  Value=Te_start
  Switch1 : Switch  Criteria=u2 > Threshold  ZeroCross=off  SaturateOnIntegerOverflow=off  InputSameDT=off
  Switch2 : Switch  Criteria=u2 > Threshold  Threshold=0.1  ZeroCross=off  SaturateOnIntegerOverflow=off  InputSameDT=off
  Switch3 : Switch  Criteria=u2 > Threshold  Threshold=10  ZeroCross=off  SaturateOnIntegerOverflow=off  InputSameDT=off
  Torque Actuator : Subsystem  mask(Torque Actuator){}
      mask help: The torque unit is Nm.
  shaft : PMIOPort  Side=Right
  wires:
  ne/1 -> Abs1/1, Switch3/2, Switch1/2
  Constant1/1 -> Switch2/3
  Switch1/1 -> Switch2/1
  Abs1/1 -> Switch2/2
  Constant3/1 -> Switch1/1
  Constant5/1 -> Switch1/3
  Constant2/1 -> Switch3/1
  Switch2/1 -> Switch3/3
  Switch3/1 -> Torque Actuator/1(torque)
  connections:
  shaft/RConn1 -- Torque Actuator/RConn1

== system EMT_ML.before_diagnostic_fixes/engine/Engine/Torque Actuator ==
  torque : Inport
  Ideal Torque Source : fl_lib/Mechanical/Mechanical Sources/Ideal Torque Source
  Mechanical Rotational Reference : fl_lib/Mechanical/Rotational Elements/Mechanical Rotational Reference
  Simulink-PS Converter : nesl_utility/Simulink-PS Converter  PhysicalDomain=network_engine_domain  SubClassName=ps_input  LeftPortType=input  RightPortType=output  PseudoPeriodic=off  Frequencies=[]  NoiseDistribution=none  NoiseParameters=[]  Unit=N*m  AffineConversion=off  FilteringAndDerivatives=filter  SimscapeFilterOrder=1  InputFilterTimeConstant=.001  UdotUserProvided=1
  shaft : PMIOPort  Side=Right
  wires:
  torque/1 -> Simulink-PS Converter/1
  connections:
  Simulink-PS Converter/RConn1 -- Ideal Torque Source/RConn1
  Mechanical Rotational Reference/LConn1 -- Ideal Torque Source/RConn2
  shaft/RConn1 -- Ideal Torque Source/LConn1

== system EMT_ML.before_diagnostic_fixes/motorA/Motor/Efficiency ==
  speed : Inport
  torque : Inport  Port=2
  Abs{,1..3} (4 alike) : Abs  SaturateOnIntegerOverflow=off
  Divide : Product  Inputs=/*
  Gain1 : Gain  Gain=1/9549
  Product1 : Product  RndMeth=Zero
  Product4 : Product  RndMeth=Zero
  Saturation : Saturate  UpperLimit=max(n_motor)  LowerLimit=min(n_motor)
  Saturation1 : Saturate  UpperLimit=max(T_motor)  LowerLimit=min(T_motor)
  Saturation2 : Saturate  UpperLimit=max(n_generator)  LowerLimit=min(n_generator)
  Saturation3 : Saturate  UpperLimit=max(T_generator)  LowerLimit=min(T_generator)
  Switch : Switch  SaturateOnIntegerOverflow=off  InputSameDT=off
  generator efficiency : Lookup2D  RowIndex=n_generator  ColumnIndex=T_generator  Table=eff_generator'  LookUpMeth=Interpolation-Use End Values  SaturateOnIntegerOverflow=off  InputSameDT=off
  motor efficiency : Lookup2D  RowIndex=n_motor  ColumnIndex=T_motor  Table=eff_motor'  LookUpMeth=Interpolation-Use End Values  SaturateOnIntegerOverflow=off  InputSameDT=off
  power : Outport
  wires:
  Abs3/1 -> Saturation3/1
  Abs2/1 -> Saturation2/1
  Abs1/1 -> Saturation1/1
  Abs/1 -> Saturation/1
  Product1/1 -> Switch/3
  generator efficiency/1 -> Product1/2
  motor efficiency/1 -> Divide/1
  Divide/1 -> Switch/1
  Saturation3/1 -> generator efficiency/2
  Saturation2/1 -> generator efficiency/1
  Saturation1/1 -> motor efficiency/2
  Saturation/1 -> motor efficiency/1
  Gain1/1 -> Switch/2, Divide/2, Product1/1
  Product4/1 -> Gain1/1
  Switch/1 -> power/1
  speed/1 -> Abs2/1, Abs/1, Product4/1
  torque/1 -> Abs3/1, Abs1/1, Product4/2

== system EMT_ML.before_diagnostic_fixes/motorA/Motor/Electrical System ==
  power : Inport
  Constant3 : Constant  Value=interp1(SOC_map,Uoc_map,SOC0)
  Controlled Current Source1 : fl_lib/Electrical/Electrical Sources/Controlled Current Source
  Divie1 : Product  Inputs=*/
  Gain : Gain  Gain=-1000
  Memory2 : Memory  InitialCondition=interp1(SOC_map,Uoc_map,SOC0)
  PS-Simulink Converter : nesl_utility/PS-Simulink Converter  PhysicalDomain=network_engine_domain  SubClassName=ps_output  LeftPortType=input  RightPortType=output  PseudoPeriodic=off  Frequencies=[]  VectorFormat=1-D array  Unit=V  AffineConversion=off
  Simulink-PS Converter : nesl_utility/Simulink-PS Converter  PhysicalDomain=network_engine_domain  SubClassName=ps_input  LeftPortType=input  RightPortType=output  PseudoPeriodic=off  Frequencies=[]  NoiseDistribution=none  NoiseParameters=[]  Unit=A  AffineConversion=off  FilteringAndDerivatives=filter  SimscapeFilterOrder=1  InputFilterTimeConstant=.001  UdotUserProvided=1
  Switch : Switch  Criteria=u2 ~= 0  SaturateOnIntegerOverflow=off  InputSameDT=off
  Voltage Sensor : fl_lib/Electrical/Electrical Sensors/Voltage Sensor
  + mot : PMIOPort  Side=Right
  - mot : PMIOPort  Port=2  Side=Right
  voltage : Outport
  wires:
  Gain/1 -> Simulink-PS Converter/1
  Memory2/1 -> Switch/1, Switch/2
  Switch/1 -> Divie1/2
  Constant3/1 -> Switch/3
  PS-Simulink Converter/1 -> voltage/1, Memory2/1
  Divie1/1 -> Gain/1
  power/1 -> Divie1/1
  connections:
  PS-Simulink Converter/LConn1 -- Voltage Sensor/RConn1
  Voltage Sensor/LConn1 -- Controlled Current Source1/LConn1 -- + mot/RConn1
  Voltage Sensor/RConn2 -- Controlled Current Source1/RConn2 -- - mot/RConn1
  Simulink-PS Converter/RConn1 -- Controlled Current Source1/RConn1

== system EMT_ML.before_diagnostic_fixes/motorA/Motor/Mechanical Body ==
  Tm_com : Inport
  Inertia1 : fl_lib/Mechanical/Rotational Elements/Inertia  inertia=Jm kg*m^2  num_ports=foundation.enum.numPorts2.one  w_specify=on  w_priority=High  w=0 rad/s  w_nominal_specify=off  w_nominal_value=1  w_nominal_unit=rad/s  t_specify=off  t_priority=None  t=0 N*m  t_nominal_specify=off  t_nominal_value=1  t_nominal_unit=N*m
  Max & Min Torque Control : Subsystem
  Memory2 : Memory
  Resistance : Subsystem
  Speed Sensor : Subsystem  mask(Speed Sensor){}
      mask help: The speed unit is r/min.
  Torque Actuator : Subsystem  mask(Torque Actuator){}
      mask help: The torque unit is Nm.
  out : PMIOPort  Side=Right
  speed : Outport
  torque : Outport  Port=2
  wires:
  Speed Sensor/1(r/min) -> Memory2/1, speed/1
  Memory2/1 -> Resistance/1(speed), Max & Min Torque Control/1(speed)
  Max & Min Torque Control/1(torque) -> Torque Actuator/1(torque), torque/1
  Tm_com/1 -> Max & Min Torque Control/2(Tm_com)
  connections:
  Inertia1/LConn1 -- Torque Actuator/RConn1 -- Resistance/RConn1 -- Speed Sensor/LConn1 -- out/RConn1

== system EMT_ML.before_diagnostic_fixes/motorB/Motor/Efficiency ==
  speed : Inport
  torque : Inport  Port=2
  Abs{,1..3} (4 alike) : Abs  SaturateOnIntegerOverflow=off
  Divide : Product  Inputs=/*
  Gain1 : Gain  Gain=1/9549
  Product1 : Product  RndMeth=Zero
  Product4 : Product  RndMeth=Zero
  Saturation : Saturate  UpperLimit=max(n_motor)  LowerLimit=min(n_motor)
  Saturation1 : Saturate  UpperLimit=max(T_motor)  LowerLimit=min(T_motor)
  Saturation2 : Saturate  UpperLimit=max(n_generator)  LowerLimit=min(n_generator)
  Saturation3 : Saturate  UpperLimit=max(T_generator)  LowerLimit=min(T_generator)
  Switch : Switch  SaturateOnIntegerOverflow=off  InputSameDT=off
  generator efficiency : Lookup2D  RowIndex=n_generator  ColumnIndex=T_generator  Table=eff_generator'  LookUpMeth=Interpolation-Use End Values  SaturateOnIntegerOverflow=off  InputSameDT=off
  motor efficiency : Lookup2D  RowIndex=n_motor  ColumnIndex=T_motor  Table=eff_motor'  LookUpMeth=Interpolation-Use End Values  SaturateOnIntegerOverflow=off  InputSameDT=off
  power : Outport
  wires:
  Abs3/1 -> Saturation3/1
  Abs2/1 -> Saturation2/1
  Abs1/1 -> Saturation1/1
  Abs/1 -> Saturation/1
  Product1/1 -> Switch/3
  generator efficiency/1 -> Product1/2
  motor efficiency/1 -> Divide/1
  Divide/1 -> Switch/1
  Saturation3/1 -> generator efficiency/2
  Saturation2/1 -> generator efficiency/1
  Saturation1/1 -> motor efficiency/2
  Saturation/1 -> motor efficiency/1
  Gain1/1 -> Switch/2, Divide/2, Product1/1
  Product4/1 -> Gain1/1
  Switch/1 -> power/1
  speed/1 -> Abs2/1, Abs/1, Product4/1
  torque/1 -> Abs3/1, Abs1/1, Product4/2

== system EMT_ML.before_diagnostic_fixes/motorB/Motor/Electrical System ==
  power : Inport
  Constant3 : Constant  Value=interp1(SOC_map,Uoc_map,SOC0)
  Controlled Current Source1 : fl_lib/Electrical/Electrical Sources/Controlled Current Source
  Divie1 : Product  Inputs=*/
  Gain : Gain  Gain=-1000
  Memory2 : Memory  InitialCondition=interp1(SOC_map,Uoc_map,SOC0)
  PS-Simulink Converter : nesl_utility/PS-Simulink Converter  PhysicalDomain=network_engine_domain  SubClassName=ps_output  LeftPortType=input  RightPortType=output  PseudoPeriodic=off  Frequencies=[]  VectorFormat=1-D array  Unit=V  AffineConversion=off
  Simulink-PS Converter : nesl_utility/Simulink-PS Converter  PhysicalDomain=network_engine_domain  SubClassName=ps_input  LeftPortType=input  RightPortType=output  PseudoPeriodic=off  Frequencies=[]  NoiseDistribution=none  NoiseParameters=[]  Unit=A  AffineConversion=off  FilteringAndDerivatives=filter  SimscapeFilterOrder=1  InputFilterTimeConstant=.001  UdotUserProvided=1
  Switch : Switch  Criteria=u2 ~= 0  SaturateOnIntegerOverflow=off  InputSameDT=off
  Voltage Sensor : fl_lib/Electrical/Electrical Sensors/Voltage Sensor
  + mot : PMIOPort  Side=Right
  - mot : PMIOPort  Port=2  Side=Right
  voltage : Outport
  wires:
  Gain/1 -> Simulink-PS Converter/1
  Memory2/1 -> Switch/1, Switch/2
  Switch/1 -> Divie1/2
  Constant3/1 -> Switch/3
  PS-Simulink Converter/1 -> voltage/1, Memory2/1
  Divie1/1 -> Gain/1
  power/1 -> Divie1/1
  connections:
  PS-Simulink Converter/LConn1 -- Voltage Sensor/RConn1
  Voltage Sensor/LConn1 -- Controlled Current Source1/LConn1 -- + mot/RConn1
  Voltage Sensor/RConn2 -- Controlled Current Source1/RConn2 -- - mot/RConn1
  Simulink-PS Converter/RConn1 -- Controlled Current Source1/RConn1

== system EMT_ML.before_diagnostic_fixes/motorB/Motor/Mechanical Body ==
  Tm_com : Inport
  Inertia1 : fl_lib/Mechanical/Rotational Elements/Inertia  inertia=Jm kg*m^2  num_ports=foundation.enum.numPorts2.one  w_specify=on  w_priority=High  w=0 rad/s  w_nominal_specify=off  w_nominal_value=1  w_nominal_unit=rad/s  t_specify=off  t_priority=None  t=0 N*m  t_nominal_specify=off  t_nominal_value=1  t_nominal_unit=N*m
  Max & Min Speed Control : Subsystem
  Memory2 : Memory
  Resistance : Subsystem
  Speed Sensor : Subsystem  mask(Speed Sensor){}
      mask help: The speed unit is r/min.
  Torque Actuator : Subsystem  mask(Torque Actuator){}
      mask help: The torque unit is Nm.
  out : PMIOPort  Side=Right
  speed : Outport
  torque : Outport  Port=2
  wires:
  Speed Sensor/1(r/min) -> Memory2/1, speed/1
  Tm_com/1 -> Max & Min Speed Control/2(Tm_com)
  Memory2/1 -> Resistance/1(speed), Max & Min Speed Control/1(speed)
  Max & Min Speed Control/1(torque) -> Torque Actuator/1(torque), torque/1
  connections:
  Speed Sensor/LConn1 -- out/RConn1 -- Torque Actuator/RConn1 -- Inertia1/LConn1 -- Resistance/RConn1

== system EMT_ML.before_diagnostic_fixes/Control Unit/Control/EVT1_H Stage/brack force ==
  Fb_com : Outport
  wires:
  [Fb_ref] -> Fb_com/1

== system EMT_ML.before_diagnostic_fixes/Control Unit/Control/EVT1_H Stage/clutches condition ==
  Mux2 : Mux
  Subsystem : Subsystem
  Subsystem1 : Subsystem
  Subsystem2 : Subsystem
  Subsystem4 : Subsystem
  clutch_com : Outport
  wires:
  Subsystem/1(C0) -> Mux2/1
  Subsystem2/1(C1) -> Mux2/4
  Subsystem1/1(Z2) -> Mux2/3
  Subsystem4/1(Z1) -> Mux2/2
  Mux2/1 -> clutch_com/1

== system EMT_ML.before_diagnostic_fixes/Control Unit/Control/EVT1_H Stage/engine swich ==
  Constant1 : Constant
  engine_swich : Outport
  wires:
  Constant1/1 -> engine_swich/1

== system EMT_ML.before_diagnostic_fixes/Control Unit/Control/EVT1_H Stage/engine torque ==
  Subsystem1 : Subsystem
  Te_com : Outport
  wires:
  [ne_act] -> Subsystem1/2(ne_act)
  [Te_ref] -> Subsystem1/1(Te_ref)
  Subsystem1/1(Te_com) -> Te_com/1

== system EMT_ML.before_diagnostic_fixes/Control Unit/Control/EVT1_H Stage/motorA torque ==
  TA_com : Outport
  wires:
  [TA_ref] -> TA_com/1

== system EMT_ML.before_diagnostic_fixes/Control Unit/Control/EVT1_H Stage/motorB torque ==
  TB_com : Outport
  wires:
  [TB_ref] -> TB_com/1

== system EMT_ML.before_diagnostic_fixes/Control Unit/Control/EVT1_H Stage/motorZ torque ==
  TZ_com : Outport
  wires:
  [TZ_ref] -> TZ_com/1

== system EMT_ML.before_diagnostic_fixes/Control Unit/Control/EVT2 Stage/brack force ==
  Fb_com : Outport
  wires:
  [Fb_ref] -> Fb_com/1

== system EMT_ML.before_diagnostic_fixes/Control Unit/Control/EVT2 Stage/clutches condition ==
  Mux2 : Mux
  Subsystem : Subsystem
  Subsystem1 : Subsystem
  Subsystem2 : Subsystem
  Subsystem4 : Subsystem
  clutch_com : Outport
  wires:
  Mux2/1 -> clutch_com/1
  Subsystem4/1(Z1) -> Mux2/2
  Subsystem1/1(Z2) -> Mux2/3
  Subsystem2/1(C1) -> Mux2/4
  Subsystem/1(C0) -> Mux2/1

== system EMT_ML.before_diagnostic_fixes/Control Unit/Control/EVT2 Stage/engine swich ==
  Constant1 : Constant
  engine_swich : Outport
  wires:
  Constant1/1 -> engine_swich/1

== system EMT_ML.before_diagnostic_fixes/Control Unit/Control/EVT2 Stage/engine torque ==
  Te_com : Outport
  wires:
  [Te_ref] -> Te_com/1

== system EMT_ML.before_diagnostic_fixes/Control Unit/Control/EVT2 Stage/motorA torque ==
  TA_com : Outport
  wires:
  [TA_ref] -> TA_com/1

== system EMT_ML.before_diagnostic_fixes/Control Unit/Control/EVT2 Stage/motorB torque ==
  TB_com : Outport
  wires:
  [TB_ref] -> TB_com/1

== system EMT_ML.before_diagnostic_fixes/Control Unit/Control/EVT2 Stage/motorZ torque ==
  Lookup Table : Lookup  InputValues=nZ_map  Table=TZ_max_map  SaturateOnIntegerOverflow=off
  Lookup Table1 : Lookup  InputValues=nZ_map  Table=TZ_min_map  SaturateOnIntegerOverflow=off
  Saturation Dynamic : simulink/Discontinuities/Saturation Dynamic  OutMin=[]  OutMax=[]  OutDataTypeStr=Inherit: Same as second input  OutDataType=sfix(16)  OutScaling=2^-10  DoSatur=off
  Saturation1 : Saturate  UpperLimit=max(nZ_map)  LowerLimit=min(nZ_map)
  Saturation2 : Saturate  UpperLimit=max(nZ_map)  LowerLimit=min(nZ_map)
  Subsystem1 : Subsystem
  TZ_com : Outport
  wires:
  Saturation Dynamic/1 -> TZ_com/1
  [nZ_act] -> Saturation1/1, Saturation2/1, Subsystem1/1(nZ_act)
  Lookup Table/1 -> Saturation Dynamic/1
  Lookup Table1/1 -> Saturation Dynamic/3
  Saturation1/1 -> Lookup Table/1
  Saturation2/1 -> Lookup Table1/1
  Subsystem1/1(TZ_com) -> Saturation Dynamic/2
